simulink model "vita_sys_05"  (R2025b)
settings: Solver=FixedStepAuto  StartTime=0.0  StopTime=10.0  RelTol=1e-3
undefined symbols (not defined in the file): matlabshared
libraries: drivingscenarioandsensors x2, drivinglib x1
settings Model: Creator=ADMIIN  LastModifiedBy=ADMIIN

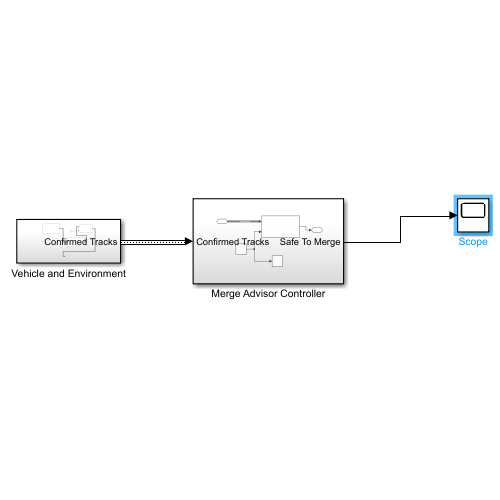
[thumbnail: Simulink's stored preview of the top-level diagram]
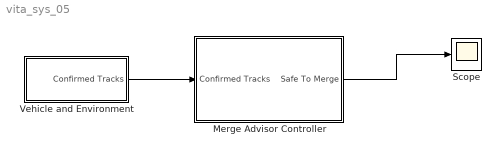
== system vita_sys_05 ==
  Merge Advisor Controller : Subsystem
  Scope : Scope
      settings: ActiveDisplayYMinimum=-1.5749885780601283  ActiveDisplayYMaximum=1.8461772208466958
  Vehicle and Environment : Subsystem
  wires:
  Vehicle and Environment/1(Confirmed Tracks) -> Merge Advisor Controller/1(Confirmed Tracks)
  Merge Advisor Controller/1(Safe To Merge) -> Scope/1

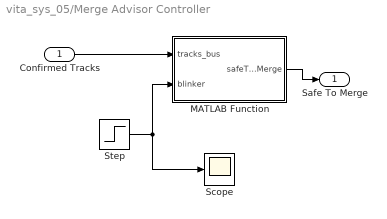
== system vita_sys_05/Merge Advisor Controller ==
  Confirmed Tracks : Inport
  MATLAB Function : MATLAB Function  TreatAsAtomicUnit=on
  Scope : Scope
      settings: ActiveDisplayYMinimum=-0.12499999999999997  ActiveDisplayYMaximum=1.125
  Step : Step  Time=4  SampleTime=0
  Safe To Merge : Outport
  wires:
  Confirmed Tracks/1 -> MATLAB Function/1(tracks_bus)
  Step/1 -> MATLAB Function/2(blinker), Scope/1
  MATLAB Function/1(safeToMerge) -> Safe To Merge/1

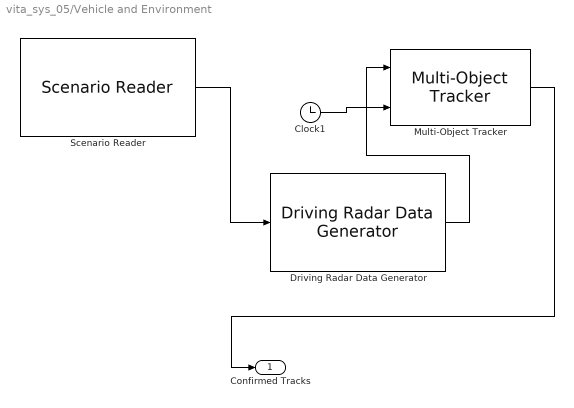
== system vita_sys_05/Vehicle and Environment ==
  Clock1 : Clock
  Driving Radar Data Generator : drivingscenarioandsensors/Driving Radar Data Generator  SensorIndex=1  UpdateRate=10  MountingLocation=[ 3.4, 0, 0.2 ]  MountingAngles=[0 0 0]  HasElevation=on  HasRangeRate=off  HasNoise=on  HasFalseAlarms=on  HasOcclusion=on  MaxNumReportsSource=Property  MaxNumReports=50  TargetReportFormat=Clustered detections  DetectionCoordinates=Body  TrackCoordinates=Body  BusNameSource=Auto  BusName=BusDrivingRadarDataGenerator  SimulateUsing=Interpreted execution  AzimuthResolution=4  ElevationResolution=5  RangeResolution=2.5  RangeRateResolution=0.5  AzimuthBiasFraction=0.1  ElevationBiasFraction=0.1  RangeBiasFraction=0.05  RangeRateBiasFraction=0.05  FieldOfView=[90, 5]  RangeLimits=[ 0, 150 ]  RangeRateLimits=[ -100, 100 ]  DetectionProbability=0.9  FalseAlarmRate=1e-06  ReferenceRange=100  ReferenceRCS=0  CenterFrequency=77e9  FilterInitializationFcn=initcvekf  ConfirmationThreshold=[2 3]  DeletionThreshold=[5 5]  InitialSeedSource=Repeatable  InitialSeed=0  UsedSeed=matlabshared.tracking.internal.SimulinkUtilities.seedManager(gcb)  ProfilesSource=From Scenario Reader block  ProfilesParameters=driving.internal.ActorProfilesRadarParameters  ProfilesExpression=struct('ClassID',0,'Length',4.7,'Width',1.8,'Height',1.4,'OriginOffset',[-1.35 0 0],'RCSPattern',[10 10;10 10],'RCSAzimuthAngles',[-180 180],'RCSElevationAngles',[-90 90])
  Multi-Object Tracker : drivinglib/Multi-Object Tracker  TrackerIndex=uint32( 0 )  FilterInitializationFcn=initcvkf  AssignmentThreshold=30.0  ConfirmationThreshold=[ 2, 3 ]  DeletionThreshold=[ 5, 5 ]  MaxNumTracks=200  MaxNumSensors=20  OOSMHandling=Neglect  StateParametersSimulink=struct  HasStateParametersInput=off  TimeInputSource=Input port  HasCostMatrixInput=off  HasDetectableTrackIDsInput=off  BusNameSource=Auto  BusName=BusMultiObjectTracker  TentativeTracksOutputPort=off  AllTracksOutputPort=off  SimulateUsing=Interpreted execution
  Scenario Reader : drivingscenarioandsensors/Scenario Reader  ScenarioSource=From file  ScenarioFileName=E:\tata\merge_scenario.mat  ScenarioVariableName=scenario  OutputCoordinateSystem=Vehicle coordinates  EgoVehicleSource=Scenario  EgoVehicleActorID=1  OrientVehiclesOnRoad=off  OutputEgoVehiclePose=off  OutputEgoVehicleState=off  SampleTime=0.1  LaneBoundaryOutput=None  LaneBoundaryDistance=0:0.5:9.5  LaneBoundaryLocation=Center of lane markings  BusNameSource=Auto  BusName=BusActors  BusNumActorsSource=Scenario  BusNumActors=100  BusName2Source=Auto  BusName2=BusLaneBoundaries  BusNumLaneBoundariesSource=Scenario  BusNumLaneBoundaries=10  BusName3Source=Auto  BusName3=BusEgoActor  BusName4Source=Auto  BusName4=BusEgoState  ShowCoordinateLabels=on  SimulateUsing=Interpreted execution
  Confirmed Tracks : Outport
  wires:
  Scenario Reader/1 -> Driving Radar Data Generator/1
  Driving Radar Data Generator/1 -> Multi-Object Tracker/1
  Multi-Object Tracker/1 -> Confirmed Tracks/1
  Clock1/1 -> Multi-Object Tracker/2

== matlab function vita_sys_05/Merge Advisor Controller/MATLAB Function ==
  data: tracks_bus input; safeToMerge output; blinker input
function safeToMerge = fcn(tracks_bus, blinker)
% This function analyzes tracks to find a safe merge gap.

% Default output
safeToMerge = 0;

% Only do the analysis if the blinker is on
if blinker == 0
    return;
end

% Safety thresholds
TIME_GAP_FOLLOWER = 3.0; % seconds
TIME_GAP_LEADER = 2.0; % seconds

% Target lane is the left lane (Y > 0)
targetLaneY = 1.85;

% Find the closest leader and follower in the target lane
closestLeaderDist = 150;
closestFollowerDist = 150;

for i = 1:tracks_bus.NumTracks
    track = tracks_bus.Tracks(i);

    % Check if the track is in the left lane
    if abs(track.State(3) - targetLaneY) < 1.8 % Is track in left lane?

        % Is it in front of us (a Leader)?
        if track.State(1) > 0 && track.State(1) < closestLeaderDist
            closestLeaderDist = track.State(1);
        end

        % Is it behind us (a Follower)?
        if track.State(1) < 0 && abs(track.State(1)) < closestFollowerDist
            closestFollowerDist = abs(track.State(1));
        end
    end
end

% Assume our speed is 25 m/s for this calculation
egoSpeed = 25;

% Calculate the time gaps
leaderGapTime = closestLeaderDist / egoSpeed;
followerGapTime = closestFollowerDist / egoSpeed;

% Apply the safety rule
if leaderGapTime > TIME_GAP_LEADER && followerGapTime > TIME_GAP_FOLLOWER
    safeToMerge = 1;
end

end
